simulink model "untitled_coder"  (R2022b)
settings: Solver=FixedStepDiscrete  StartTime=0.0  StopTime=0.03  FixedStep=5e-05  RelTol=1e-3
undefined symbols (not defined in the file or in its folder): motor, obs, pll, sim
settings Model: Creator=17850  LastModifiedBy=17850
settings OptimizationCC: DefaultParameterBehavior=Inlined  EnhancedBackFolding=on  PassReuseOutputArgsAs=Individual arguments  ZeroExternalMemoryAtStartup=off  ZeroInternalMemoryAtStartup=off  OptimizeBlockOrder=speed  DifferentSizesBufferReuse=on  OptimizationCustomize=off  EfficientTunableParamExpr=on
settings DebuggingCC: ParameterTunabilityLossMsg=error
settings SFSimCC: MATLABDynamicMemAlloc=off
settings RTWCC: Description=Embedded Coder  SystemTargetFile=ert.tlc  TemplateMakefile=ert_default_tmf  GenerateReport=on  LaunchReport=on
settings CodeAppCC: ForceParamTrailComments=on  IgnoreCustomStorageClasses=off  OperatorAnnotations=on  SimulinkDataObjDesc=on  SFDataObjDesc=on  InsertBlockDesc=on
settings ERTTargetCC: TargetLangStandard=C99 (ISO)  GenerateSampleERTMain=on  InlinedParameterPlacement=NonHierarchical  ERTCustomFileTemplate=example_file_process.tlc

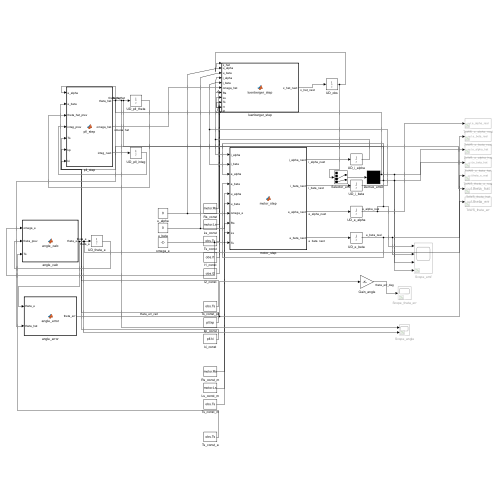
[thumbnail: Simulink's stored preview of the top-level diagram]
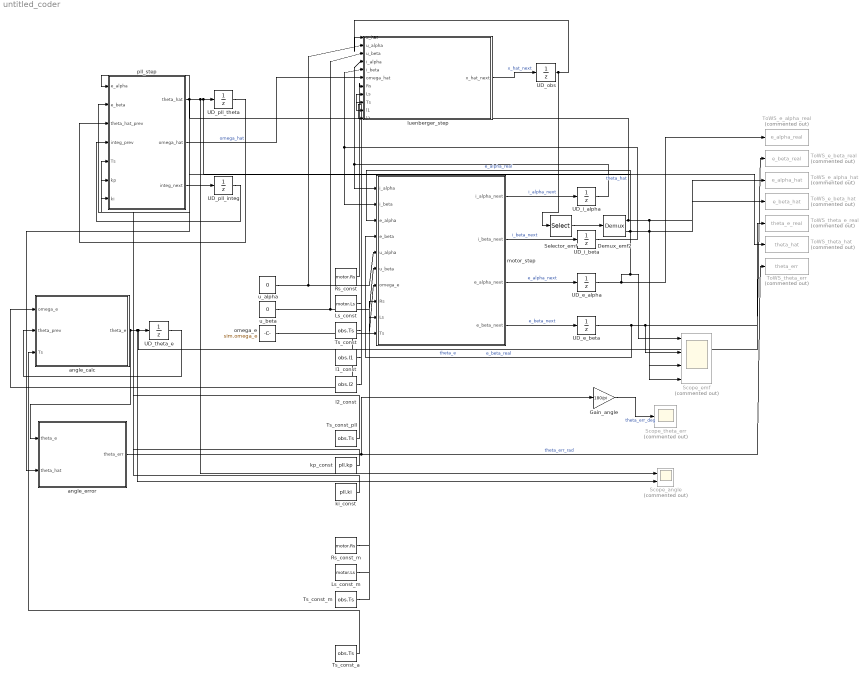
== system untitled_coder ==
  Demux_emf2 : Demux  Outputs=2
  Gain_angle : Gain  Gain=180/pi
  Ls_const : Constant  Value=motor.Ls
  Ls_const_m : Constant  Value=motor.Ls
  Rs_const : Constant  Value=motor.Rs
  Rs_const_m : Constant  Value=motor.Rs
  Scope_angle : Scope  Commented=on  NumInputPorts=2
  Scope_emf : Scope  Commented=on  NumInputPorts=4
  Scope_theta_err : Scope  Commented=on
  Selector_emf : Selector  IndexMode=Zero-based  InputPortWidth=4  IndexOptions=Index vector (dialog)  Indices=[2 3]  OutputSizes=1
  ToWS_e_alpha_hat : ToWorkspace  Commented=on  VariableName=e_alpha_hat  SaveFormat=Structure With Time  SampleTime=-1
  ToWS_e_alpha_real : ToWorkspace  Commented=on  VariableName=e_alpha_real  SaveFormat=Structure With Time  SampleTime=-1
  ToWS_e_beta_hat : ToWorkspace  Commented=on  VariableName=e_beta_hat  SaveFormat=Structure With Time  SampleTime=-1
  ToWS_e_beta_real : ToWorkspace  Commented=on  VariableName=e_beta_real  SaveFormat=Structure With Time  SampleTime=-1
  ToWS_theta_e_real : ToWorkspace  Commented=on  VariableName=theta_e_real  SaveFormat=Structure With Time  SampleTime=-1
  ToWS_theta_err : ToWorkspace  Commented=on  VariableName=theta_err  SaveFormat=Structure With Time  SampleTime=-1
  ToWS_theta_hat : ToWorkspace  Commented=on  VariableName=theta_hat  SaveFormat=Structure With Time  SampleTime=-1
  Ts_const : Constant  Value=obs.Ts
  Ts_const_a : Constant  Value=obs.Ts
  Ts_const_m : Constant  Value=obs.Ts
  Ts_const_pll : Constant  Value=obs.Ts
  UD_e_alpha : UnitDelay  InitialCondition=1  SampleTime=obs.Ts  HasFrameUpgradeWarning=on
  UD_e_beta : UnitDelay  SampleTime=obs.Ts  HasFrameUpgradeWarning=on
  UD_i_alpha : UnitDelay  SampleTime=obs.Ts  HasFrameUpgradeWarning=on
  UD_i_beta : UnitDelay  SampleTime=obs.Ts  HasFrameUpgradeWarning=on
  UD_obs : UnitDelay  InitialCondition=[0;0;0;0]  SampleTime=obs.Ts  HasFrameUpgradeWarning=on
  UD_pll_integ : UnitDelay  SampleTime=obs.Ts  HasFrameUpgradeWarning=on
  UD_pll_theta : UnitDelay  SampleTime=obs.Ts  HasFrameUpgradeWarning=on
  UD_theta_e : UnitDelay  InitialCondition=-pi/2  SampleTime=obs.Ts  HasFrameUpgradeWarning=on
  angle_calc : MATLAB Function  TreatAsAtomicUnit=on
  angle_error : MATLAB Function  TreatAsAtomicUnit=on
  ki_const : Constant  Value=pll.ki
  kp_const : Constant  Value=pll.kp
  l1_const : Constant  Value=obs.l1
  l2_const : Constant  Value=obs.l2
  luenberger_step : MATLAB Function  TreatAsAtomicUnit=on
  motor_step : MATLAB Function  TreatAsAtomicUnit=on
  omega_e : Constant  Value=sim.omega_e
  pll_step : MATLAB Function  TreatAsAtomicUnit=on
  u_alpha : Constant  Value=0
  u_beta : Constant  Value=0
  wires:
  luenberger_step/1(x_hat_next) -> UD_obs/1  "x_hat_next"
  UD_obs/1 -> luenberger_step/1(x_hat), Selector_emf/1
  pll_step/1(theta_hat) -> ToWS_theta_hat/1, UD_pll_theta/1, Scope_angle/1, angle_error/2(theta_hat)  "theta_hat"
  UD_pll_theta/1 -> pll_step/3(theta_hat_prev)
  pll_step/3(integ_next) -> UD_pll_integ/1
  UD_pll_integ/1 -> pll_step/4(integ_prev)
  pll_step/2(omega_hat) -> luenberger_step/6(omega_hat)  "omega_hat"
  motor_step/1(i_alpha_next) -> UD_i_alpha/1  "i_alpha_next"
  motor_step/2(i_beta_next) -> UD_i_beta/1  "i_beta_next"
  motor_step/3(e_alpha_next) -> UD_e_alpha/1  "e_alpha_next"
  motor_step/4(e_beta_next) -> UD_e_beta/1  "e_beta_next"
  omega_e/1 -> angle_calc/1(omega_e), motor_step/7(omega_e)
  u_alpha/1 -> luenberger_step/2(u_alpha), motor_step/5(u_alpha)
  u_beta/1 -> luenberger_step/3(u_beta), motor_step/6(u_beta)
  UD_i_alpha/1 -> luenberger_step/4(i_alpha), motor_step/1(i_alpha)
  UD_i_beta/1 -> luenberger_step/5(i_beta), motor_step/2(i_beta)
  UD_e_alpha/1 -> motor_step/3(e_alpha), Scope_emf/1, ToWS_e_alpha_real/1  "e_alpha_real"
  UD_e_beta/1 -> ToWS_e_beta_real/1, Scope_emf/2, motor_step/4(e_beta)  "e_beta_real"
  angle_calc/1(theta_e) -> ToWS_theta_e_real/1, UD_theta_e/1, Scope_angle/2, angle_error/1(theta_e)  "theta_e"
  UD_theta_e/1 -> angle_calc/2(theta_prev)
  angle_error/1(theta_err) -> Gain_angle/1, ToWS_theta_err/1  "theta_err_rad"
  Gain_angle/1 -> Scope_theta_err/1  "theta_err_deg"
  Selector_emf/1 -> Demux_emf2/1
  Demux_emf2/1 -> Scope_emf/3, ToWS_e_alpha_hat/1, pll_step/1(e_alpha)
  Demux_emf2/2 -> Scope_emf/4, ToWS_e_beta_hat/1, pll_step/2(e_beta)
  Rs_const/1 -> luenberger_step/7(Rs)
  Ls_const/1 -> luenberger_step/8(Ls)
  Ts_const/1 -> luenberger_step/9(Ts)
  l1_const/1 -> luenberger_step/10(l1)
  l2_const/1 -> luenberger_step/11(l2)
  Ts_const_pll/1 -> pll_step/5(Ts)
  kp_const/1 -> pll_step/6(kp)
  ki_const/1 -> pll_step/7(ki)
  Rs_const_m/1 -> motor_step/8(Rs)
  Ls_const_m/1 -> motor_step/9(Ls)
  Ts_const_m/1 -> motor_step/10(Ts)
  Ts_const_a/1 -> angle_calc/3(Ts)

== matlab function untitled_coder/pll_step ==
  data: e_alpha input; theta_hat output; e_beta input; theta_hat_prev input; integ_prev input; omega_hat output; integ_next output; Ts input; kp input; ki input
function [theta_hat, omega_hat, integ_next] = pll_step(e_alpha, e_beta, theta_hat_prev, integ_prev, Ts, kp, ki)
    e_alpha = e_alpha(1);
    e_beta  = e_beta(1);

    epsilon = -e_alpha*cos(theta_hat_prev) - e_beta*sin(theta_hat_prev);

    omega_hat = kp*epsilon + integ_prev;
    integ_next = integ_prev + Ts*ki*epsilon;
    theta_hat = mod(theta_hat_prev + Ts*omega_hat, 2*pi);
end

== matlab function untitled_coder/luenberger_step ==
  data: x_hat input; x_hat_next output; u_alpha input; u_beta input; i_alpha input; i_beta input; omega_hat input; Rs input; Ls input; Ts input; l1 input; l2 input
function x_hat_next = luenberger_step(x_hat, u_alpha, u_beta, i_alpha, i_beta, omega_hat, Rs, Ls, Ts, l1, l2)
    i_alpha_hat = x_hat(1);
    i_beta_hat  = x_hat(2);
    e_alpha_hat = x_hat(3);
    e_beta_hat  = x_hat(4);

    di_alpha = (-Rs/Ls)*i_alpha_hat - (1/Ls)*e_alpha_hat + (1/Ls)*u_alpha + l1*(i_alpha - i_alpha_hat);
    di_beta  = (-Rs/Ls)*i_beta_hat  - (1/Ls)*e_beta_hat  + (1/Ls)*u_beta  + l1*(i_beta  - i_beta_hat);

    i_alpha_hat_next = i_alpha_hat + Ts*di_alpha;
    i_beta_hat_next  = i_beta_hat  + Ts*di_beta;

    theta = omega_hat * Ts;
    R = [cos(theta), -sin(theta); sin(theta), cos(theta)];
    e_rot = R * [e_alpha_hat; e_beta_hat];
    e_alpha_hat_next = e_rot(1) + Ts*(-l2)*(i_alpha - i_alpha_hat);
    e_beta_hat_next  = e_rot(2) + Ts*(-l2)*(i_beta  - i_beta_hat);

    x_hat_next = [i_alpha_hat_next; i_beta_hat_next; e_alpha_hat_next; e_beta_hat_next];
end

== matlab function untitled_coder/motor_step ==
  data: i_alpha input; i_alpha_next output; i_beta input; e_alpha input; e_beta input; u_alpha input; u_beta input; omega_e input; i_beta_next output; e_alpha_next output; e_beta_next output; Rs input; Ls input; Ts input
function [i_alpha_next, i_beta_next, e_alpha_next, e_beta_next] = motor_step(i_alpha, i_beta, e_alpha, e_beta, u_alpha, u_beta, omega_e, Rs, Ls, Ts)
    di_alpha = (-Rs/Ls)*i_alpha - (1/Ls)*e_alpha + (1/Ls)*u_alpha;
    di_beta  = (-Rs/Ls)*i_beta  - (1/Ls)*e_beta  + (1/Ls)*u_beta;

    i_alpha_next = i_alpha + Ts*di_alpha;
    i_beta_next  = i_beta  + Ts*di_beta;

    theta = omega_e * Ts;
    R = [cos(theta), -sin(theta); sin(theta), cos(theta)];
    e_rot = R * [e_alpha; e_beta];
    e_alpha_next = e_rot(1);
    e_beta_next  = e_rot(2);
end

== matlab function untitled_coder/angle_calc ==
  data: omega_e input; theta_e output; theta_prev input; Ts input
function theta_e = angle_calc(omega_e, theta_prev, Ts)
    theta_e = mod(theta_prev + Ts*omega_e, 2*pi);
end

== matlab function untitled_coder/angle_error ==
  data: theta_e input; theta_err output; theta_hat input
function theta_err = angle_error(theta_e, theta_hat)
    theta_err = mod(theta_e - theta_hat + pi, 2*pi) - pi;
end
